simulink model "lazo_camara_l3"  (R2024b)
settings: Solver=ode4  StartTime=0.0  StopTime=TF  FixedStep=T/NSUB  RelTol=1e-3
values from neighbouring files (symbols this model uses):
  bias_g = 0.5*D2R    (= 0.00872664625997)    [simulink_lazo_camara_l3.m]
  D2R = pi/180    (= 0.0174532925199)    [simulink_lazo_camara_l3.m]
  DZ_HAT = 0    [simulink_lazo_camara_l3.m]    (also in tst_004_pwm_actuador.m = dzh)
  Kc = 30    [simulink_lazo_camara_l3.m]
  Kc_hat = Kc    (= 30)    [simulink_lazo_camara_l3.m]
  l1 = 2*ze*we    (= 0.7)    [simulink_lazo_camara_l3.m]
  l2 = we^2    (= 0.25)    [simulink_lazo_camara_l3.m]
  psi0 = psib_data(1, 2) + 1.5*D2R    [simulink_lazo_camara_l3.m]    (also in tst_004_pwm_actuador.m)
  psib0 = psib_data(1, 2)    [simulink_lazo_camara_l3.m]    (also in tst_004_pwm_actuador.m)
  PWM_BITS = Inf    (= inf)    [simulink_lazo_camara_l3.m]    (also in tst_004_pwm_actuador.m = nb)
  R = conv([1 x(1)], [1 -1])    [simulink_lazo_camara_l3.m]
  S = x(2:4)'    [simulink_lazo_camara_l3.m]
  sig_g = 0.1*D2R    (= 0.00174532925199)    [simulink_lazo_camara_l3.m]
  sig_m = 0.9*D2R    (= 0.0157079632679)    [simulink_lazo_camara_l3.m]
  T = 0.01    [simulink_lazo_camara_l3.m]
  tau = 0.1    [simulink_lazo_camara_l3.m]
  Tp = Km*Ao    [simulink_lazo_camara_l3.m]
  U_DZ = 0    [simulink_lazo_camara_l3.m]    (also in tst_004_pwm_actuador.m = udz)
  UMAX = 6    [simulink_lazo_camara_l3.m]
  VBAT = 7.4    [simulink_lazo_camara_l3.m]    (also in tst_004_pwm_actuador.m = vb)
  VBAT_HAT = 7.4    [simulink_lazo_camara_l3.m]    (also in tst_004_pwm_actuador.m = vbh)
  wb0 = wb_data(1, 2)    [simulink_lazo_camara_l3.m]    (also in tst_004_pwm_actuador.m)
settings Model: Creator=angelrevelo  LastModifiedBy=angelrevelo
settings DataIOCC: SaveOutput=off  SaveTime=off

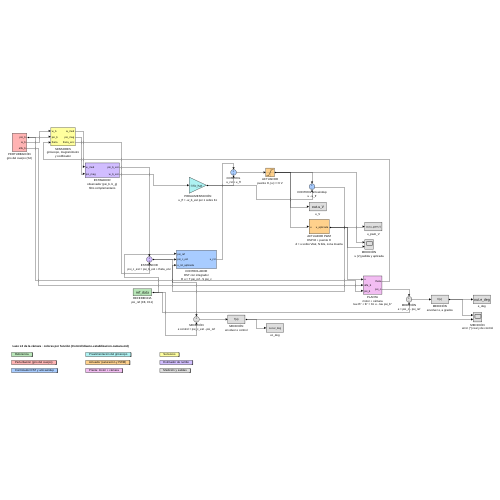
[thumbnail: Simulink's stored preview of the top-level diagram]
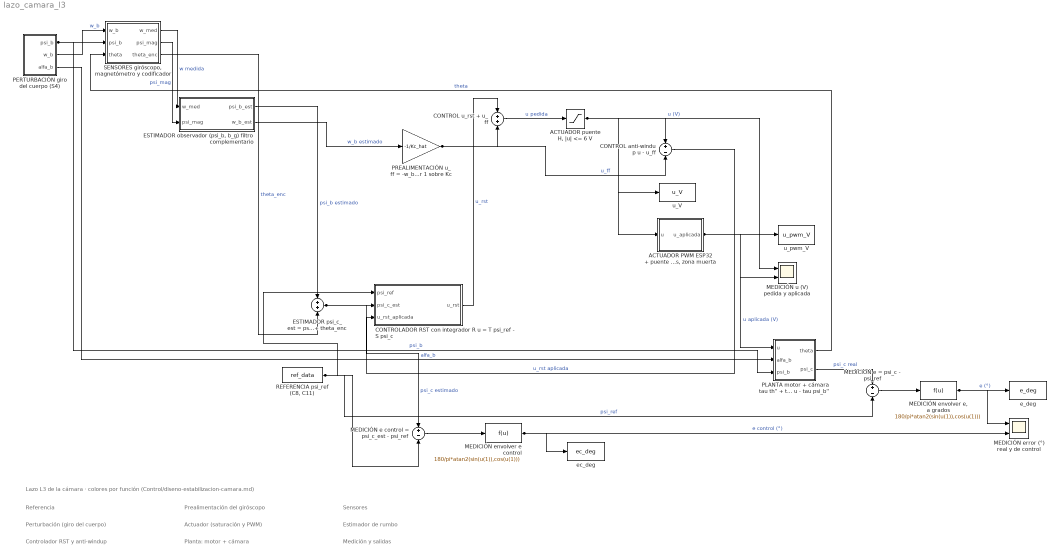
== system lazo_camara_l3 ==
  note: Lazo L3 de la cámara · colores por función (Control/diseno-estabilizacion-camara.md)
  note: Referencia
  note: Perturbación (giro del cuerpo)
  note: Controlador RST y anti-windup
  note: Prealimentación del giróscopo
  note: Actuador (saturación y PWM)
  note: Planta: motor + cámara
  note: Sensores
  note: Estimador de rumbo
  note: Medición y salidas
  "ACTUADOR puente H, |u| <= 6 V" : Saturate  UpperLimit=UMAX  LowerLimit=-UMAX
  "ACTUADOR PWM ESP32 + puente H d = u sobre Vbat, N bits, zona muerta" : Subsystem
  CONTROL u_rst + u_ff : Sum
  CONTROL anti-windup u - u_ff : Sum  Inputs=+-
  CONTROLADOR RST con integrador R u = T psi_ref - S psi_c : Subsystem
  "ESTIMADOR observador (psi_b, b_g) filtro complementario" : Subsystem
  ESTIMADOR psi_c_est = psi_b_est + theta_enc : Sum
  MEDICIÓN e = psi_c - psi_ref : Sum  Inputs=+-
  MEDICIÓN e control = psi_c_est - psi_ref : Sum  Inputs=+-
  MEDICIÓN envolver e control : Fcn  Expr=180/pi*atan2(sin(u(1)),cos(u(1)))
  "MEDICIÓN envolver e, a grados" : Fcn  Expr=180/pi*atan2(sin(u(1)),cos(u(1)))
  MEDICIÓN error (°) real y de control : Scope  NumInputPorts=2
  MEDICIÓN u (V) pedida y aplicada : Scope  NumInputPorts=2
  PERTURBACIÓN giro del cuerpo (S4) : Subsystem
  PLANTA motor + cámara tau th'' + th' = Kc u - tau psi_b'' : Subsystem
  PREALIMENTACIÓN u_ff = -w_b_est por 1 sobre Kc : Gain  Gain=-1/Kc_hat
  "REFERENCIA psi_ref (C8, C11)" : FromWorkspace  VariableName=ref_data  OutputAfterFinalValue=Holding final value
  "SENSORES giróscopo, magnetómetro y codificador" : Subsystem
  e_deg : ToWorkspace  VariableName=e_deg  SaveFormat=Timeseries  SampleTime=T
  ec_deg : ToWorkspace  VariableName=ec_deg  SaveFormat=Timeseries  SampleTime=T
  u_V : ToWorkspace  VariableName=u_V  SaveFormat=Timeseries  SampleTime=T
  u_pwm_V : ToWorkspace  VariableName=u_pwm_V  SaveFormat=Timeseries  SampleTime=T
  wires:
  PLANTA motor + cámara tau th'' + th' = Kc u - tau psi_b''/2(psi_c) -> MEDICIÓN e = psi_c - psi_ref/1  "psi_c real"
  PLANTA motor + cámara tau th'' + th' = Kc u - tau psi_b''/1(theta) -> "SENSORES giróscopo, magnetómetro y codificador"/3(theta)  "theta"
  "ACTUADOR puente H, |u| <= 6 V"/1 -> u_V/1, "ACTUADOR PWM ESP32 + puente H d = u sobre Vbat, N bits, zona muerta"/1(u), MEDICIÓN u (V) pedida y aplicada/1, CONTROL anti-windup u - u_ff/1  "u (V)"
  MEDICIÓN envolver e control/1 -> ec_deg/1, MEDICIÓN error (°) real y de control/2  "e control (°)"
  CONTROL u_rst + u_ff/1 -> "ACTUADOR puente H, |u| <= 6 V"/1  "u pedida"
  PERTURBACIÓN giro del cuerpo (S4)/1(psi_b) -> "SENSORES giróscopo, magnetómetro y codificador"/2(psi_b), PLANTA motor + cámara tau th'' + th' = Kc u - tau psi_b''/3(psi_b)  "psi_b"
  MEDICIÓN e = psi_c - psi_ref/1 -> "MEDICIÓN envolver e, a grados"/1
  CONTROLADOR RST con integrador R u = T psi_ref - S psi_c/1(u_rst) -> CONTROL u_rst + u_ff/1  "u_rst"
  PERTURBACIÓN giro del cuerpo (S4)/3(alfa_b) -> PLANTA motor + cámara tau th'' + th' = Kc u - tau psi_b''/2(alfa_b)  "alfa_b"
  "SENSORES giróscopo, magnetómetro y codificador"/1(w_med) -> "ESTIMADOR observador (psi_b, b_g) filtro complementario"/1(w_med)  "w medida"
  "ESTIMADOR observador (psi_b, b_g) filtro complementario"/1(psi_b_est) -> ESTIMADOR psi_c_est = psi_b_est + theta_enc/1  "psi_b estimado"
  CONTROL anti-windup u - u_ff/1 -> CONTROLADOR RST con integrador R u = T psi_ref - S psi_c/3(u_rst_aplicada)  "u_rst aplicada"
  PREALIMENTACIÓN u_ff = -w_b_est por 1 sobre Kc/1 -> CONTROL u_rst + u_ff/2, CONTROL anti-windup u - u_ff/2  "u_ff"
  "SENSORES giróscopo, magnetómetro y codificador"/2(psi_mag) -> "ESTIMADOR observador (psi_b, b_g) filtro complementario"/2(psi_mag)  "psi_mag"
  "MEDICIÓN envolver e, a grados"/1 -> e_deg/1, MEDICIÓN error (°) real y de control/1  "e (°)"
  MEDICIÓN e control = psi_c_est - psi_ref/1 -> MEDICIÓN envolver e control/1
  PERTURBACIÓN giro del cuerpo (S4)/2(w_b) -> "SENSORES giróscopo, magnetómetro y codificador"/1(w_b)  "w_b"
  "SENSORES giróscopo, magnetómetro y codificador"/3(theta_enc) -> ESTIMADOR psi_c_est = psi_b_est + theta_enc/2  "theta_enc"
  "ESTIMADOR observador (psi_b, b_g) filtro complementario"/2(w_b_est) -> PREALIMENTACIÓN u_ff = -w_b_est por 1 sobre Kc/1  "w_b estimado"
  "ACTUADOR PWM ESP32 + puente H d = u sobre Vbat, N bits, zona muerta"/1(u_aplicada) -> u_pwm_V/1, MEDICIÓN u (V) pedida y aplicada/2, PLANTA motor + cámara tau th'' + th' = Kc u - tau psi_b''/1(u)  "u aplicada (V)"
  ESTIMADOR psi_c_est = psi_b_est + theta_enc/1 -> CONTROLADOR RST con integrador R u = T psi_ref - S psi_c/2(psi_c_est), MEDICIÓN e control = psi_c_est - psi_ref/1  "psi_c estimado"
  "REFERENCIA psi_ref (C8, C11)"/1 -> CONTROLADOR RST con integrador R u = T psi_ref - S psi_c/1(psi_ref), MEDICIÓN e = psi_c - psi_ref/2, MEDICIÓN e control = psi_c_est - psi_ref/2  "psi_ref"

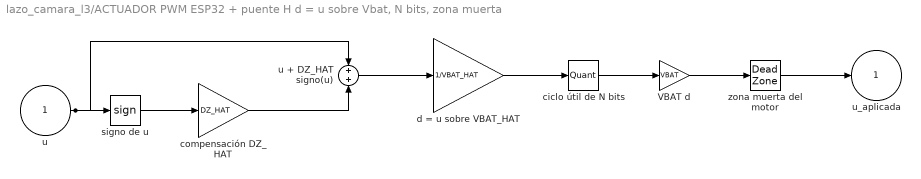
== system lazo_camara_l3/ACTUADOR PWM ESP32 + puente H d = u sobre Vbat, N bits, zona muerta ==
  u : Inport
  VBAT d : Gain  Gain=VBAT
  ciclo útil de N bits : Quantizer  QuantizationInterval=max(2^-PWM_BITS, eps)
  compensación DZ_HAT : Gain  Gain=DZ_HAT
  d = u sobre VBAT_HAT : Gain  Gain=1/VBAT_HAT
  signo de u : Signum
  u + DZ_HAT signo(u) : Sum
  zona muerta del motor : DeadZone  LowerValue=-U_DZ  UpperValue=U_DZ
  u_aplicada : Outport
  wires:
  VBAT d/1 -> zona muerta del motor/1
  ciclo útil de N bits/1 -> VBAT d/1
  d = u sobre VBAT_HAT/1 -> ciclo útil de N bits/1
  u + DZ_HAT signo(u)/1 -> d = u sobre VBAT_HAT/1
  zona muerta del motor/1 -> u_aplicada/1
  compensación DZ_HAT/1 -> u + DZ_HAT signo(u)/2
  signo de u/1 -> compensación DZ_HAT/1
  u/1 -> signo de u/1, u + DZ_HAT signo(u)/1

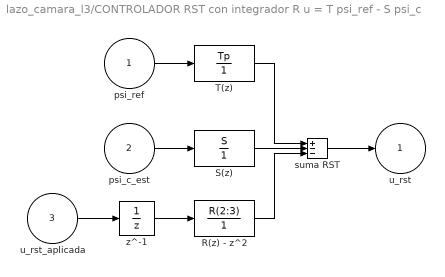
== system lazo_camara_l3/CONTROLADOR RST con integrador R u = T psi_ref - S psi_c ==
  psi_ref : Inport
  psi_c_est : Inport  Port=2
  u_rst_aplicada : Inport  Port=3
  R(z) - z^2 : DiscreteFilter  Numerator=R(2:3)  Denominator=1  SampleTime=T
  S(z) : DiscreteFilter  Numerator=S  Denominator=1  SampleTime=T
  T(z) : DiscreteFilter  Numerator=Tp  Denominator=1  SampleTime=T
  suma RST : Sum  Inputs=+--
  z^-1 : UnitDelay  SampleTime=T  HasFrameUpgradeWarning=on
  u_rst : Outport
  wires:
  suma RST/1 -> u_rst/1
  S(z)/1 -> suma RST/2
  T(z)/1 -> suma RST/1
  z^-1/1 -> R(z) - z^2/1
  R(z) - z^2/1 -> suma RST/3
  psi_c_est/1 -> S(z)/1
  psi_ref/1 -> T(z)/1
  u_rst_aplicada/1 -> z^-1/1

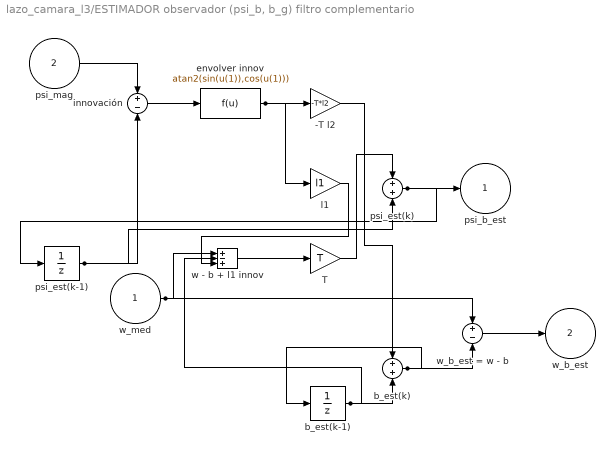
== system lazo_camara_l3/ESTIMADOR observador (psi_b, b_g) filtro complementario ==
  w_med : Inport
  psi_mag : Inport  Port=2
  -T l2 : Gain  Gain=-T*l2
  T : Gain  Gain=T
  b_est(k) : Sum
  b_est(k-1) : UnitDelay  SampleTime=T  HasFrameUpgradeWarning=on
  envolver innov : Fcn  Expr=atan2(sin(u(1)),cos(u(1)))
  innovación : Sum  Inputs=+-
  l1 : Gain  Gain=l1
  psi_est(k) : Sum
  psi_est(k-1) : UnitDelay  InitialCondition=psi0  SampleTime=T  HasFrameUpgradeWarning=on
  w - b + l1 innov : Sum  Inputs=+-+
  w_b_est = w - b : Sum  Inputs=+-
  psi_b_est : Outport
  w_b_est : Outport  Port=2
  wires:
  w_b_est = w - b/1 -> w_b_est/1
  b_est(k)/1 -> w_b_est = w - b/2, b_est(k-1)/1
  T/1 -> psi_est(k)/1
  l1/1 -> w - b + l1 innov/3
  -T l2/1 -> b_est(k)/1
  w - b + l1 innov/1 -> T/1
  b_est(k-1)/1 -> b_est(k)/2, w - b + l1 innov/2
  envolver innov/1 -> -T l2/1, l1/1
  w_med/1 -> w - b + l1 innov/1, w_b_est = w - b/1
  psi_est(k)/1 -> psi_b_est/1, psi_est(k-1)/1
  innovación/1 -> envolver innov/1
  psi_est(k-1)/1 -> innovación/2, psi_est(k)/2
  psi_mag/1 -> innovación/1

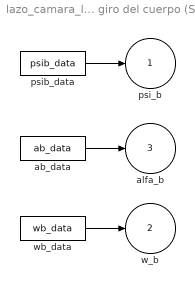
== system lazo_camara_l3/PERTURBACIÓN giro del cuerpo (S4) ==
  ab_data : FromWorkspace  VariableName=ab_data  OutputAfterFinalValue=Holding final value
  psib_data : FromWorkspace  VariableName=psib_data  OutputAfterFinalValue=Holding final value
  wb_data : FromWorkspace  VariableName=wb_data  OutputAfterFinalValue=Holding final value
  psi_b : Outport
  w_b : Outport  Port=2
  alfa_b : Outport  Port=3
  wires:
  wb_data/1 -> w_b/1
  ab_data/1 -> alfa_b/1
  psib_data/1 -> psi_b/1

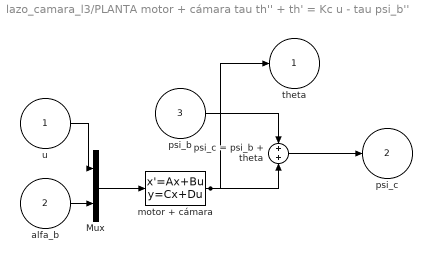
== system lazo_camara_l3/PLANTA motor + cámara tau th'' + th' = Kc u - tau psi_b'' ==
  u : Inport
  alfa_b : Inport  Port=2
  psi_b : Inport  Port=3
  Mux : Mux  Inputs=2
  motor + cámara : StateSpace  A=[0 1; 0 -1/tau]  B=[0 0; Kc/tau -1]  C=[1 0]  D=[0 0]  InitialCondition=0
  psi_c = psi_b + theta : Sum
  theta : Outport
  psi_c : Outport  Port=2
  wires:
  psi_c = psi_b + theta/1 -> psi_c/1
  motor + cámara/1 -> theta/1, psi_c = psi_b + theta/2
  psi_b/1 -> psi_c = psi_b + theta/1
  Mux/1 -> motor + cámara/1
  alfa_b/1 -> Mux/2
  u/1 -> Mux/1

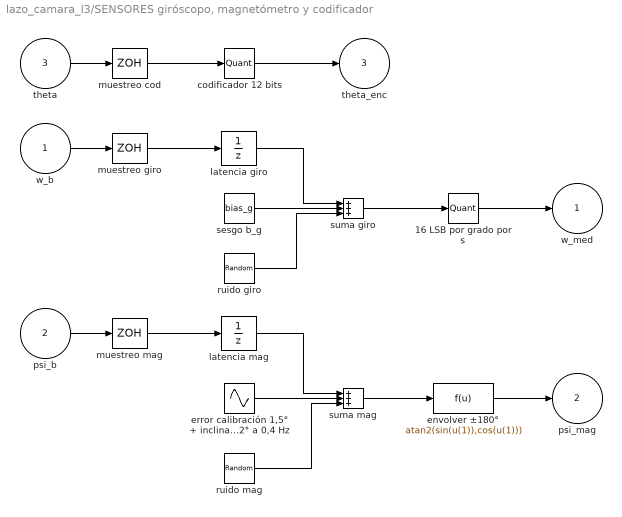
== system lazo_camara_l3/SENSORES giróscopo, magnetómetro y codificador ==
  w_b : Inport
  psi_b : Inport  Port=2
  theta : Inport  Port=3
  16 LSB por grado por s : Quantizer  QuantizationInterval=q_g
  codificador 12 bits : Quantizer  QuantizationInterval=q_enc
  envolver ±180° : Fcn  Expr=atan2(sin(u(1)),cos(u(1)))
  error calibración 1,5° + inclinación 2° a 0,4 Hz : Sin  Amplitude=2*D2R  Bias=1.5*D2R  Frequency=2*pi*0.4  SampleTime=T
  latencia giro : UnitDelay  InitialCondition=wb0  SampleTime=T  HasFrameUpgradeWarning=on
  latencia mag : UnitDelay  InitialCondition=psib0  SampleTime=T  HasFrameUpgradeWarning=on
  muestreo cod : ZeroOrderHold  SampleTime=T
  muestreo giro : ZeroOrderHold  SampleTime=T
  muestreo mag : ZeroOrderHold  SampleTime=T
  ruido giro : RandomNumber  Variance=sig_g^2  Seed=101  SampleTime=T
  ruido mag : RandomNumber  Variance=sig_m^2  Seed=102  SampleTime=T
  sesgo b_g : Constant  Value=bias_g  SampleTime=T
  suma giro : Sum  Inputs=+++
  suma mag : Sum  Inputs=+++
  w_med : Outport
  psi_mag : Outport  Port=2
  theta_enc : Outport  Port=3
  wires:
  envolver ±180°/1 -> psi_mag/1
  16 LSB por grado por s/1 -> w_med/1
  suma giro/1 -> 16 LSB por grado por s/1
  w_b/1 -> muestreo giro/1
  psi_b/1 -> muestreo mag/1
  muestreo cod/1 -> codificador 12 bits/1
  muestreo giro/1 -> latencia giro/1
  muestreo mag/1 -> latencia mag/1
  theta/1 -> muestreo cod/1
  codificador 12 bits/1 -> theta_enc/1
  ruido giro/1 -> suma giro/3
  ruido mag/1 -> suma mag/3
  latencia giro/1 -> suma giro/1
  sesgo b_g/1 -> suma giro/2
  latencia mag/1 -> suma mag/1
  suma mag/1 -> envolver ±180°/1
  error calibración 1,5° + inclinación 2° a 0,4 Hz/1 -> suma mag/2
